simulink model "Ch15Ex2"  (Simulink 4.00)
settings: Solver=ode45  StartTime=0.0  StopTime=50  RelTol=1e-3

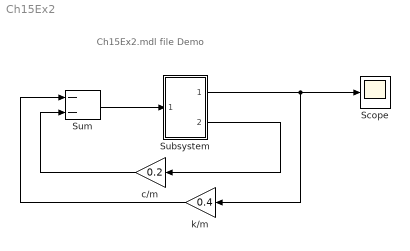
== system Ch15Ex2 ==
  note: Ch15Ex2.mdl file Demo
  Scope : Scope
      settings: TimeRange=auto  YMin=-5  YMax=5  SaveToWorkspace=off  SaveName=ScopeData  LimitDataPoints=on  MaxDataPoints=5000
  Subsystem : Subsystem
      settings: RTWFcnNameOpts=Auto  RTWFileNameOpts=Auto
  Sum : Sum  Inputs=--  SaturateOnIntegerOverflow=on
  c/m : Gain  Orientation=left  Gain=0.2  Multiplication=Element-wise(K.*u)  SaturateOnIntegerOverflow=on
  k/m : Gain  Orientation=left  Gain=0.4  Multiplication=Element-wise(K.*u)  SaturateOnIntegerOverflow=on
  wires:
  Sum/1 -> Subsystem/1(In1)
  c/m/1 -> Sum/2
  k/m/1 -> Sum/1
  Subsystem/1(Out1) -> k/m/1, Scope/1
  Subsystem/2(Out2) -> c/m/1

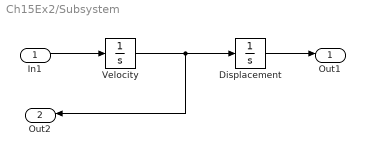
== system Ch15Ex2/Subsystem ==
  In1 : Inport  Port=1  LatchInput=off
  Displacement : Integrator  ExternalReset=none  InitialConditionSource=internal  InitialCondition=1  LimitOutput=off  UpperSaturationLimit=inf  LowerSaturationLimit=-inf  ShowSaturationPort=off  ShowStatePort=off  AbsoluteTolerance=auto
  Velocity : Integrator  ExternalReset=none  InitialConditionSource=internal  InitialCondition=0  LimitOutput=off  UpperSaturationLimit=inf  LowerSaturationLimit=-inf  ShowSaturationPort=off  ShowStatePort=off  AbsoluteTolerance=auto
  Out1 : Outport  Port=1
  Out2 : Outport  Orientation=left  Port=2
  wires:
  Velocity/1 -> Displacement/1, Out2/1
  In1/1 -> Velocity/1
  Displacement/1 -> Out1/1
